simulink model "ADCSSimulator"  (R2024a)
settings: Solver=ode4  StartTime=0.0  StopTime=600  FixedStep=0.01  MaxStep=0.1  RelTol=1e-3  AbsTol=1e-3
values from neighbouring files (symbols this model uses):
  ActuatorAllocationMatrix = ActuatorPhysicalMatrix' * inv(ActuatorPhysicalMatrix * ActuatorPhysicalMatrix')    [set_Init.m]
  ActuatorPhysicalMatrix = [1, 0, 0, 0 ... (first row only)    [set_Init.m]
  albedo_irradiance = 300    [set_Init.m]
  b = 0    [set_Init.m]
  Cd = 2.2    [set_Init.m]
  h_bias = [0; 0; 0]    [set_Init.m]
  J = 4.0e-3 / 628    (= 6.36942675159e-06)    [set_Init.m]
  k_Bdot = ((4 * pi * 0.5236 * 0.0055) / (5677.2 * (4.5e-5)^2))    (= 3147.8423197)    [set_Init.m]
  K_E = K_T    (= 0.0022)    [set_Init.m]
  K_T = 0.0022    [set_Init.m]
  P0 = blkdiag(P0_att, P0_bias)    [set_Init.m]
  P0_att = eye(3) * initial_variance_rad2    [set_Init.m]
  PowerVoltageBus_01 = 3.3    [set_Init.m]
  PowerVoltageBus_02 = 3.3    [set_Init.m]
  PowerVoltageBus_03 = 3.3    [set_Init.m]
  PowerVoltageBus_04 = 3.3    [set_Init.m]
  PowerVoltageBus_05 = 3.3    [set_Init.m]
  PowerVoltageBus_06 = 3.3    [set_Init.m]
  PowerVoltageBus_07 = 3.3    [set_Init.m]
  PowerVoltageBus_08 = 3.3    [set_Init.m]
  PowerVoltageBus_09 = 3.3    [set_Init.m]
  PowerVoltageBus_10 = 3.3    [set_Init.m]
  PowerVoltageBus_11 = 3.3    [set_Init.m]
  PowerVoltageBus_12 = 0.0    (= 0)    [set_Init.m]
  PowerVoltageBus_13 = 0.0    (= 0)    [set_Init.m]
  PowerVoltageBus_14 = 0.0    (= 0)    [set_Init.m]
  PowerVoltageBus_15 = 0.0    (= 0)    [set_Init.m]
  R = 2.0    (= 2)    [set_Init.m]
  ressidual_m = [3e-4; -2e-4; 1e-4]    [set_Init.m]
  solar_irradiance = 1361    [set_Init.m]
  surface_areas = [A_xy, A_yz, A_xz, A_xy, A_yz, A_xz]    [set_Init.m]
  surface_normals_body = [eye(3) -eye(3)]    [set_Init.m]
  surface_positions_body = [       hx,   0,   0 ... (first row only)    [set_Init.m]
  surface_reflectivities = [0.9 0.8 0.9 0.9 0.9 0.9]    [set_Init.m]
  Switch_01 = 1    [set_Init.m]
  Switch_02 = 1    [set_Init.m]
  Switch_03 = 1    [set_Init.m]
  Switch_04 = 1    [set_Init.m]
  Switch_05 = 1    [set_Init.m]
  Switch_06 = 1    [set_Init.m]
  Switch_07 = 1    [set_Init.m]
  Switch_08 = 1    [set_Init.m]
  Switch_09 = 1    [set_Init.m]
  Switch_10 = 1    [set_Init.m]
  Switch_11 = 1    [set_Init.m]
  Switch_12 = 0    [set_Init.m]
  Switch_13 = 0    [set_Init.m]
  Switch_14 = 0    [set_Init.m]
  Switch_15 = 0    [set_Init.m]
  visSampleTime = 0.1    [set_Init.m]
undefined symbols (not defined in the file or in its folder): attitude, Controller, epoch, IAU, juliandate, Kd, km, Kp, m, rad, s, satellite, SGP4_parameters, simulator, UKF_parameters, WMM2020
libraries: sharedtransform x27, aerolibutil x22, aerolibconvert2 x18, simulink_extras x16, matrix_library x6, aerolibtransform2 x4, vrlib x2, aerolibgravity2 x2, aerolibobsolete x1, aerolibattitudesys x1, simulink x1
(part 8 of 8)

== matlab function ADCSSimulator/ADCS/ADCS Software/Orbit Detemination/UKF Orbit  ==
  data: is_reset_triggered input; initial_state input; initial_covariance input; gps_pos_ICRF input; r_est_ICRF output; dt input; Q input; R input; v_est_ICRF output; Bc_est output; satellite_mass_kg input; P_out output; is_healthy output
function [r_est_ICRF, v_est_ICRF, Bc_est, P_out, is_healthy] = ukf_orbit_estimator(is_reset_triggered, initial_state, initial_covariance, gps_pos_ICRF, dt, Q, R, satellite_mass_kg)
% ukf_orbit_estimator Estimates satellite orbit state using a 7-state UKF.
%
% Function Objective:
% This function is the primary, high-fidelity orbit estimator. It fuses a
% physics-based dynamics model with GPS measurements to produce an accurate
% and continuously updated state estimate. It includes a health flag to
% enable system-level fault detection.
%
% Key Features:
%   - 7-State Vector: [r, v, Bc] for adaptive drag estimation.
%   - Reset Mechanism: Allows re-initialization from a TLE.
%   - Health Monitoring: Outputs a flag indicating filter health.
%   - Advanced Dynamics: Includes J2 and atmospheric drag.
%
% Inputs:
%   is_reset_triggered: (boolean)  If true, reset filter to initial values.
%   initial_state:      (7x1 double) State for initialization [r, v, Bc].
%   initial_covariance: (7x7 double) Covariance for initialization.
%   gps_pos_ICRF:       (3x1 double) GPS position in ICRF [km]. Use NaN if invalid.
%   dt:                 (double)   Time step [s].
%   Q:                  (7x7 double) Process noise covariance.
%   R:                  (3x3 double) Measurement noise covariance.
%   satellite_mass_kg:  (double)   Satellite mass [kg].
%
% Outputs:
%   r_est_ICRF: (3x1 double) Estimated position [km].
%   v_est_ICRF: (3x1 double) Estimated velocity [km/s].
%   Bc_est:     (double)   Estimated ballistic coefficient [m^2/kg].
%   P_out:      (7x7 double) Final estimated covariance.
%   is_healthy: (boolean)  True if the filter is operating correctly.
%===============================================================================

    persistent x_est P;

    % --- Initialization and Reset Logic ---
    if isempty(x_est) || is_reset_triggered
        x_est = initial_state;
        P = initial_covariance;
    end

    % --- UKF Tuning Parameters ---
    n = 7; alpha = 1e-3; kappa = 0; beta = 2;
    lambda = alpha^2 * (n + kappa) - n;

    %===========================================================================
    % --- 1. PREDICTION STEP ---
    %===========================================================================
    sigma_points = zeros(n, 2*n + 1);
    sigma_points(:, 1) = x_est;
    
    % --- Cholesky Decomposition for Sigma Points ---
    % This is a critical health check. If P is not positive definite, the
    % filter has mathematically diverged.
    [P_sqrt, p] = chol((n + lambda) * P, 'lower');
    if p > 0
        % CRITICAL FAILURE: Report unhealthy and exit immediately.
        r_est_ICRF = x_est(1:3); v_est_ICRF = x_est(4:6);
        Bc_est = x_est(7); P_out = P;
        is_healthy = false; % This flag triggers the switch to SAFE mode.
        return;
    end
    
    for i = 1:n
        sigma_points(:, i+1)   = x_est + P_sqrt(:, i);
        sigma_points(:, i+n+1) = x_est - P_sqrt(:, i);
    end

    % --- Propagate Sigma Points through Non-Linear Dynamics ---
    propagated_sigma_points = zeros(n, 2*n + 1);
    for i = 1:(2*n + 1)
        propagated_sigma_points(:, i) = state_transition_function(sigma_points(:, i), dt, satellite_mass_kg);
    end

    % --- Calculate Predicted State and Covariance ---
    weights_m = [lambda/(n+lambda), 0.5/(n+lambda) * ones(1, 2*n)];
    weights_c = weights_m;
    weights_c(1) = weights_c(1) + (1 - alpha^2 + beta);
    
    x_priori = propagated_sigma_points * weights_m';
    
    P_priori = zeros(n, n);
    for i = 1:(2*n + 1)
        diff = propagated_sigma_points(:, i) - x_priori;
        P_priori = P_priori + weights_c(i) * (diff * diff');
    end
    P_priori = P_priori + Q;

    %===========================================================================
    % --- 2. UPDATE STEP ---
    %===========================================================================
    if ~any(isnan(gps_pos_ICRF))
        % Transform sigma points into measurement space (position only)
        z_sigma_points = propagated_sigma_points(1:3, :);
        z_pred = z_sigma_points * weights_m';

        % Calculate Innovation Covariance (S) and Cross-Covariance (T)
        S = zeros(3, 3); T = zeros(n, 3);
        for i = 1:(2*n + 1)
            z_diff = z_sigma_points(:, i) - z_pred;
            x_diff = propagated_sigma_points(:, i) - x_priori;
            S = S + weights_c(i) * (z_diff * z_diff');
            T = T + weights_c(i) * (x_diff * z_diff');
        end
        S = S + R;
        
        % Calculate Kalman Gain and update state/covariance
        K = T / S;
        innovation = gps_pos_ICRF - z_pred;
        x_est = x_priori + K * innovation;
        P = P_priori - K * S * K';
    else
        % No GPS data, so the prediction becomes the best estimate
        x_est = x_priori;
        P = P_priori;
    end
    
    % Enforce physical constraint on the ballistic coefficient
    if x_est(7) < 0, x_est(7) = 0; end

    % --- Final Output ---
    r_est_ICRF = x_est(1:3);
    v_est_ICRF = x_est(4:6);
    Bc_est     = x_est(7);
    P_out      = P;
    is_healthy = true; % If we reached this point, the filter is healthy.
end

% --- Sub-function: State Transition (Dynamics Integration) ---
function x_next = state_transition_function(x, dt, m)
    k1 = dynamics(x, m);
    k2 = dynamics(x + 0.5*dt*k1, m);
    k3 = dynamics(x + 0.5*dt*k2, m);
    k4 = dynamics(x + dt*k3, m);
    x_next = x + (dt/6)*(k1 + 2*k2 + 2*k3 + k4);
end

% --- Sub-function: Equations of Motion ---
function dxdt = dynamics(x, m)
    r_vec = x(1:3); v_vec = x(4:6); Bc = x(7);
    r_norm = norm(r_vec);
    
    % --- Physical Constants ---
    mu = 398600.4418; J2 = 0.00108263; R_earth = 6378.137;
    
    % --- Gravitational Model ---
    a_2body = -mu * r_vec / r_norm^3;
    pre = -1.5 * mu * J2 * R_earth^2 / r_norm^5;
    z_factor = 5 * (r_vec(3)/r_norm)^2;
    a_j2 = [pre * r_vec(1) * (1 - z_factor);
            pre * r_vec(2) * (1 - z_factor);
            pre * r_vec(3) * (3 - z_factor)];
            
    % --- Atmospheric Drag Model ---
    alt_km = r_norm - R_earth;
    rho = atmospheric_density_model(alt_km); % kg/m^3
    
    we = 7.292115e-5; % Earth rotation rate [rad/s]
    v_rel_m_s = (v_vec - cross([0; 0; we], r_vec)) * 1000; % to m/s
    v_rel_norm = norm(v_rel_m_s);
    
    a_drag_m_s2 = -0.5 * Bc * rho * v_rel_norm * v_rel_m_s;
    a_drag_km_s2 = a_drag_m_s2 / 1000; % to km/s^2
    
    a_total = a_2body + a_j2 + a_drag_km_s2;
    
    % The derivative of Bc is modeled as zero (a random walk)
    dxdt = [v_vec; a_total; 0];
end

% --- Sub-function: Atmospheric Density Model ---
function rho = atmospheric_density_model(alt_km)
    % Simple exponential atmospheric density model.
    % NOTE: For a high-fidelity thesis, replacing this with a standard model
    % (e.g., NRLMSISE-00) would be a major enhancement.
    h0 = 400; rho0 = 2.4e-12; H = 55;
    rho = rho0 * exp(-(alt_km - h0) / H);
end

== matlab function ADCSSimulator/ADCS/ADCS Software/Attitude Determination/Attitude Estimation Algorithm (MEKF)/MATLAB Function9 ==
  data: q_est output; P_est output; q_feedback input; P_feedback input; q_quest input; P_quest_attitude input; lambda_max_quest input; gyro_meas input; b_sun input; b_mag input; r_sun input; r_mag input; dt input; Q_noise input; R_sun input; R_mag input; reset_threshold input
function [q_est, P_est] = attitude_mekf_simplified( ...
    q_feedback, P_feedback, ...
    q_quest, P_quest_attitude, lambda_max_quest, ...
    gyro_meas, b_sun, b_mag, r_sun, r_mag, ...
    dt, Q_noise, R_sun, R_mag, reset_threshold)
% ATTITUDE_EKF_SIMPLIFIED (Quaternion Estimation Only)
%
% This is a simplified, robust MEKF that only estimates the attitude.
% It uses a safe initialization and robustly hybridizes with QUEST
% solutions when they are available and of high quality.
%
% UNIT CONVENTION
% Attitude Error State & Covariance: milli-radians (mrad)
% Gyro Measurement:                milli-radians/second (mrad/s)
% Magnetic Field Measurement:      micro-Tesla (uT)
%
% Sun Sensor Noise R_sun:          radians^2 (rad^2)
% Mag Sensor Noise R_mag:          micro-Tesla^2 (uT^2)
% Process Noise Q_noise (3x3):     (mrad/s)^2
% =========================================================================
% 0) INITIALIZATION & HYBRIDIZATION
% =========================================================================
LAMBDA_THRESHOLD = 0.999;
is_sun_available = ~any(isnan(b_sun));
is_quest_valid = is_sun_available && ~any(isnan(q_quest)) && (lambda_max_quest > LAMBDA_THRESHOLD);

% Check if this is the first run of the simulation
is_first_run = (norm(q_feedback) < 1e-6);

if is_first_run
    % On the first run, ALWAYS initialize with a default attitude and
    % a very large uncertainty to ensure a safe start.
    q_prev = [1; 0; 0; 0];
    P_prev = eye(3) * 1e9; % Huge uncertainty: (1e6 mrad)^2
else
    % Standard Operation: Check for Reset
    perform_reset = false;
    if is_quest_valid
        % Only reset if the MEKF is more uncertain than a fresh QUEST solution
        if trace(P_feedback) > trace(P_quest_attitude) && trace(P_feedback) > reset_threshold
            perform_reset = true;
        end
    end

    if perform_reset
        % Reset the state using the high-quality QUEST solution
        q_prev = q_quest;
        P_prev = P_quest_attitude;
    else
        % No reset, continue propagating the filter's own estimate
        q_prev = q_feedback;
        P_prev = P_feedback;
    end
end

% =========================================================================
% 1) PREDICTION
% =========================================================================
omega = gyro_meas; % No bias estimation
q_pred = propagate_with_gyro_expmap(q_prev, omega, dt);

% State is 3x1 (d_theta), so Fx is 3x3
Fx = -skew_symmetric(omega / 1000); % Convert mrad/s to rad/s for kinematics
F = expm(Fx * dt);

P_pred = F * P_prev * F' + Q_noise;
P_pred = 0.5 * (P_pred + P_pred'); % Enforce symmetry

% =========================================================================
% 2) BATCH UPDATE
% =========================================================================
q_est = q_pred;
P_est = P_pred;

H_stack = zeros(6,3);
y_stack = zeros(6,1);
R_stack = zeros(6,6);
num_valid = 0;
C_pred = quat2rotm(q_pred');

% Sun Sensor Measurement
if is_sun_available
    num_valid = num_valid + 1;
    idx = 1:3;
    b_pred_sun = C_pred * r_sun;
    y_sun      = b_sun - b_pred_sun;
    H_sun      = skew_symmetric(b_pred_sun) / 1000; % Maps d(theta)_mrad to d(y)_rad

    H_stack(idx,:) = H_sun;
    y_stack(idx)   = y_sun;
    R_stack(idx,idx) = R_sun;
end

% Magnetometer Measurement
if ~any(isnan(b_mag))
    num_valid = num_valid + 1;
    idx = (num_valid-1)*3 + (1:3);
    b_pred_mag = C_pred * r_mag;
    y_mag      = b_mag - b_pred_mag;
    H_mag      = skew_symmetric(b_pred_mag) / 1000; % Maps d(theta)_mrad to d(y)_uT

    H_stack(idx,:)   = H_mag;
    y_stack(idx)     = y_mag;
    R_stack(idx,idx) = R_mag;
end

% Perform Update
if num_valid > 0
    m = num_valid*3;
    H = H_stack(1:m,:);
    y = y_stack(1:m,:);
    R = R_stack(1:m,1:m);

    S = H*P_pred*H' + R;
    S = 0.5*(S + S');

    K = (P_pred*H') / S;

    dtheta_mrad = K * y;
    dtheta_rad = dtheta_mrad / 1000;

    dq = [1; 0.5*dtheta_rad];
    dq = dq / norm(dq);

    q_est = quat_multiply(q_pred, dq);

    I_KH = eye(3) - K*H;
    P_est = I_KH*P_pred*I_KH' + K*R*K';
    P_est = 0.5*(P_est + P_est');
end

q_est = q_est / norm(q_est);

end

% =========================================================================
% Helper Functions
% =========================================================================
function q_out = propagate_with_gyro_expmap(q_prev, omega_mrad_s, dt)
    omega_rad_s = omega_mrad_s / 1000;
    theta = norm(omega_rad_s) * dt;
    if theta > 1e-9
        axis = omega_rad_s / (theta/dt);
        half = 0.5*theta;
        dq = [cos(half); axis * sin(half)];
        q_out = quat_multiply(q_prev, dq);
    else
        q_out = q_prev;
    end
    q_out = q_out / norm(q_out);
end

function C = skew_symmetric(v)
    C = [   0   -v(3)  v(2);
          v(3)    0   -v(1);
         -v(2)  v(1)    0  ];
end

function q_out = quat_multiply(q1, q2)
    w1 = q1(1); v1 = q1(2:4);
    w2 = q2(1); v2 = q2(2:4);
    w  = w1*w2 - dot(v1,v2);
    v  = w1*v2 + w2*v1 + cross(v1,v2);
    q_out = [w; v];
end

== matlab function ADCSSimulator/ADCS/ADCS Software/MATLAB Function2 ==
  data: p input; trace_p output
function trace_p = Trace(p)

trace_p = trace(p);

== matlab function ADCSSimulator/ADCS/ADCS Software/Orbit Detemination/UKF Orbit Estimator ==
  settings: updateMethod=DISCRETE
  data: r_meas input; r_est output; dt input; v_est output; Q input; R input; P_out output
function [r_est, v_est, P_out] = ukf_orbit_simple(r_meas, dt, Q, R)
% UKF orbit estimator (position only as measurement)
% 6-state UKF: [r; v]

persistent x_est P

n = 6; alpha = 1e-3; kappa = 0; beta = 2;
lambda = alpha^2*(n+kappa)-n;

% Initialize persistent state
if isempty(x_est)
    x_est = [r_meas; zeros(3,1)];
    P = eye(6)*1e4;
end

% Sigma points
sigma_pts = zeros(n,2*n+1);
sigma_pts(:,1) = x_est;
[P_sqrt, p] = chol((n+lambda)*P,'lower');
if p>0
    P_sqrt = sqrt(n+lambda)*eye(n);
end
for i=1:n
    sigma_pts(:,i+1)   = x_est + P_sqrt(:,i);
    sigma_pts(:,i+n+1) = x_est - P_sqrt(:,i);
end

% Propagate sigma points
prop_sigma = zeros(n,2*n+1);
for i=1:2*n+1
    prop_sigma(:,i) = rk4_orbit(sigma_pts(:,i), dt);
end

% Predicted state and covariance
wm = [lambda/(n+lambda) repmat(0.5/(n+lambda),1,2*n)];
wc = wm; wc(1) = wc(1)+(1-alpha^2+beta);

x_priori = prop_sigma*wm';
P_priori = zeros(n);
for i=1:2*n+1
    diff = prop_sigma(:,i)-x_priori;
    P_priori = P_priori + wc(i)*(diff*diff');
end
P_priori = P_priori + Q;

% Measurement update
if ~any(isnan(r_meas))
    Z = prop_sigma(1:3,:);
    z_pred = Z*wm';
    
    S = zeros(3); T = zeros(n,3);
    for i=1:2*n+1
        dz = Z(:,i)-z_pred;
        dx = prop_sigma(:,i)-x_priori;
        S = S + wc(i)*(dz*dz');
        T = T + wc(i)*(dx*dz');
    end
    S = S + R;
    K = T/S;
    x_est = x_priori + K*(r_meas - z_pred);
    P = P_priori - K*S*K';
else
    x_est = x_priori;
    P = P_priori;
end

r_est = x_est(1:3);
v_est = x_est(4:6);
P_out = P;

end

%% RK4 integrator
function x_next = rk4_orbit(x, dt)
r = x(1:3); v = x(4:6);

k1 = orbit_dynamics(r,v);
k2 = orbit_dynamics(r + 0.5*dt*k1(1:3), v + 0.5*dt*k1(4:6));
k3 = orbit_dynamics(r + 0.5*dt*k2(1:3), v + 0.5*dt*k2(4:6));
k4 = orbit_dynamics(r + dt*k3(1:3), v + dt*k3(4:6));

r_next = r + dt/6*(k1(1:3)+2*k2(1:3)+2*k3(1:3)+k4(1:3));
v_next = v + dt/6*(k1(4:6)+2*k2(4:6)+2*k3(4:6)+k4(4:6));

x_next = [r_next; v_next];
end

%% Orbital dynamics (gravity + J2)
function dx = orbit_dynamics(r,v)
mu = 3.986004418e14; Re = 6378137; J2 = 1.08263e-3;
r_norm = norm(r);
a_grav = -mu*r/r_norm^3;

% J2 perturbation
rx=r(1); ry=r(2); rz=r(3); z2=rz^2;
fac = 1.5*J2*mu*Re^2/r_norm^5;
a_j2 = fac * [rx*(5*z2/r_norm^2 - 1); ry*(5*z2/r_norm^2 - 1); rz*(5*z2/r_norm^2 -3)];

dx = [v; a_grav + a_j2];
end

== matlab function ADCSSimulator/ADCS/ADCS Software/Attitude Control/Chart/Nadir_Pointing/َAttitude Controller (LQR Controller)/PD Quaternion Feedback Controller/Dipole Smoother00 ==
  data: B input; m output; T_c input; k input
function m = computeMagneticDipole(B, T_c, k)
    % Computes the magnetic dipole moment (m) given:
    % B: Geomagnetic field vector in body frame [3x1] (T)
    % Tc: Commanded control torque in body frame [3x1] (N·m)
    % k: Regularization constant (scalar)
    %
    % Output:
    % m: Magnetic dipole moment in body frame [3x1] (A·m^2)

    % Validate inputs
    if length(B) ~= 3 || length(T_c) ~= 3
        error('B and Tc must be 3x1 vectors.');
    end

    % Create the skew-symmetric matrix of B
    B_mat = [
        0,       B(3),  -B(2);
       -B(3),   0,       B(1);
        B(2),  -B(1),    0
    ];

    % Compute the SR-Inverse
    I = eye(3); % 3x3 identity matrix
    regularized_inverse = inv((B_mat.' * B_mat + k * I)) / B_mat.';

    % Compute the magnetic dipole moment
    m = regularized_inverse * T_c;
end

== matlab function ADCSSimulator/ADCS/ADCS Software/Orbit Detemination/Mode Manager2 ==
  data: r_true input; error_vec output; r_est input; RMS_error output; mean_error output
function [error_vec, RMS_error, mean_error] = evaluate_position_error(r_true, r_est)
% evaluate_position_error Computes the estimation error of satellite position
%
% Inputs:
%   r_true - Nx3 matrix of true satellite positions [m]
%   r_est  - Nx3 matrix of estimated satellite positions [m]
%
% Outputs:
%   error_vec  - Nx1 vector of position errors (Euclidean distance) [m]
%   RMS_error  - Root-mean-square error over all samples [m]
%   mean_error - Mean absolute error over all samples [m]

    % Ensure same size
    if size(r_true,1) ~= size(r_est,1)
        error('r_true and r_est must have the same number of samples.');
    end

    % Vector of Euclidean errors
    error_vec = sqrt(sum((r_true - r_est).^2, 2));

    % RMS error
    RMS_error = sqrt(mean(error_vec.^2));

    % Mean absolute error
    mean_error = mean(error_vec);
end

== matlab function ADCSSimulator/ADCS/ADCS Software/Orbit Detemination/UKF Orbit Estimator1 ==
  data: gps_pos_ICRF input; r_est output; dt input; v_est output; Q_in input; R_in input; init_flag input; x0 input; P0 input; P_out output; is_healthy output
function [r_est, v_est, P_out, is_healthy] = ukf_orbit_block(gps_pos_ICRF, dt, Q_in, R_in, init_flag, x0, P0)
% UKF_ORBIT_BLOCK - 6-state UKF for ICRF orbit (2-body + J2 + drag + SRP)
% Inputs:
%  gps_pos_ICRF : 3x1 measured position [m] (use NaN to skip update)
%  dt            : timestep [s]
%  Q_in          : 6x6 process noise covariance (optional; pass [] to use default)
%  R_in          : 3x3 measurement noise covariance (optional; pass [] to use default)
%  init_flag     : boolean, true => initialize with x0 and P0
%  x0            : 6x1 initial state [r0; v0] (required if init_flag true)
%  P0            : 6x6 initial covariance (optional)
% Outputs:
%  r_est, v_est, P_out, is_healthy

    persistent x_est P params ukf_initialized

    % -------------------- default physical params (SI) --------------------
    if isempty(params)
        params.mu     = 3.986004418e14;   % m^3/s^2
        params.Re     = 6378137.0;        % m
        params.J2     = 1.08263e-3;
        params.omegaE = 7.2921150e-5;     % rad/s

        % CubeSat example
        params.m  = 4.0;   % kg
        params.A  = 0.03;  % m^2
        params.Cd = 2.2;
        params.Cr = 1.3;

        % SRP
        params.Psrp  = 4.56e-6;           % N/m^2
        params.r_sun = [1.496e11; 0; 0];  % approx 1 AU along +x

        % atmosphere exponential baseline (around 400 km)
        params.rho0 = 2.4e-12;  % kg/m^3 at h0
        params.h0   = 400e3;    % m
        params.H    = 55e3;     % m
    end

    % -------------------- defaults for Q, R, P0 --------------------
    default_P0 = diag([100^2,100^2,100^2, 0.1^2,0.1^2,0.1^2]);
    default_Q  = diag([1e-4,1e-4,1e-4, 1e-8,1e-8,1e-8]);
    default_R  = diag([15^2,15^2,15^2]);

    if isempty(Q_in)
        Q = default_Q;
    else
        Q = Q_in;
    end
    if isempty(R_in)
        R = default_R;
    else
        R = R_in;
    end

    % -------------------- UKF tuning --------------------
    n = 6;
    alpha = 1e-2; beta = 2; kappa = 0;
    lambda = alpha^2*(n + kappa) - n;
    c = n + lambda;
    Wm = zeros(2*n+1,1); Wc = zeros(2*n+1,1);
    Wm(1) = lambda / c; Wc(1) = Wm(1) + (1 - alpha^2 + beta);
    Wm(2:end) = 1/(2*c); Wc(2:end) = 1/(2*c);

    % -------------------- initialization --------------------
    if isempty(ukf_initialized) || init_flag
        if init_flag
            if nargin < 6 || isempty(x0) || numel(x0)~=6
                error('init_flag true requires x0 (6x1).');
            end
            x_est = x0(:);
        else
            % first call without explicit init -> try init from gps_pos_ICRF
            if any(isnan(gps_pos_ICRF))
                error('First call requires valid gps_pos_ICRF or init_flag=true with x0.');
            end
            r0 = gps_pos_ICRF(:);
            rnorm = norm(r0) + 1e-12;
            % approximate circular speed and direction (tangent)
            vmag = sqrt(params.mu / rnorm);
            % choose a stable perpendicular vector
            k = [0;0;1];
            t = cross(k, r0);
            if norm(t) < 1e-6
                t = cross([1;0;0], r0);
            end
            t = t / norm(t);
            v0 = vmag * t;
            x_est = [r0; v0];
        end
        if nargin>=7 && ~isempty(P0)
            P = P0;
        else
            P = default_P0;
        end
        ukf_initialized = true;
    end

    is_healthy = true;

    % -------------------- ensure shapes --------------------
    gps_pos_ICRF = gps_pos_ICRF(:);
    if numel(gps_pos_ICRF)~=3
        error('gps_pos_ICRF must be 3x1 (or NaN).');
    end

    % -------------------- 1) sigma points --------------------
    P = 0.5*(P + P.');  % symmetrize
    try
        A = chol(c * P, 'lower'); % A*A' = cP
    catch
        % regularize and retry
        epsfix = 1e-9 * eye(n);
        try
            A = chol(c * (P + epsfix), 'lower');
        catch
            % catastrophic -> soft reset if measurement available
            is_healthy = false;
            if ~any(isnan(gps_pos_ICRF))
                % reinit with measurement pos and approximate vel
                r0 = gps_pos_ICRF(:);
                rnorm = norm(r0) + 1e-12;
                vmag = sqrt(params.mu / rnorm);
                k = [0;0;1];
                t = cross(k, r0);
                if norm(t) < 1e-6, t = cross([1;0;0], r0); end
                t = t / norm(t);
                x_est = [r0; vmag*t];
                P = default_P0;
                r_est = x_est(1:3); v_est = x_est(4:6); P_out = P;
                return
            else
                r_est = x_est(1:3); v_est = x_est(4:6); P_out = P;
                return
            end
        end
    end

    X = zeros(n, 2*n+1);
    X(:,1) = x_est;
    for i=1:n
        X(:,i+1)   = x_est + A(:,i);
        X(:,i+1+n) = x_est - A(:,i);
    end

    % -------------------- 2) propagate sigma points (RK4) --------------------
    Xprop = zeros(size(X));
    for i=1:size(X,2)
        Xprop(:,i) = propagate_rk4(X(:,i), dt, params);
    end

    % -------------------- 3) predicted mean & covariance --------------------
    x_pred = Xprop * Wm;
    P_pred = zeros(n);
    for i=1:2*n+1
        dx = Xprop(:,i) - x_pred;
        P_pred = P_pred + Wc(i) * (dx * dx.');
    end
    P_pred = P_pred + Q;

    % -------------------- 4) measurement update (position only) --------------------
    if ~any(isnan(gps_pos_ICRF))
        z = gps_pos_ICRF(:);
        Zsig = Xprop(1:3, :);
        z_pred = Zsig * Wm;

        S = zeros(3);
        Pxz = zeros(n,3);
        for i=1:2*n+1
            dz = Zsig(:,i) - z_pred;
            dx = Xprop(:,i) - x_pred;
            S = S + Wc(i) * (dz * dz.');
            Pxz = Pxz + Wc(i) * (dx * dz.');
        end
        S = S + R;

        % Kalman gain
        K = Pxz / S;
        innov = z - z_pred;

        % gating (simple)
        nis = innov' * (S\innov);
        gating_thresh = 16; % ~ chi2inv(0.995,3) ~ 12.84 ; use small margin
        if nis > 1e6
            % catastrophic innovation: skip update, mark unhealthy
            x_est = x_pred;
            P = P_pred;
            is_healthy = false;
        elseif nis > gating_thresh
            % large innovation: reject update (keep prediction)
            x_est = x_pred;
            P = P_pred;
            is_healthy = false;
        else
            x_est = x_pred + K * innov;
            P = P_pred - K * S * K.';
        end
    else
        x_est = x_pred;
        P = P_pred;
    end

    % -------------------- postprocess P --------------------
    P = 0.5*(P + P.');
    % small eigen-clamp to remove numerical negative eigenvalues
    [V,D] = eig(P);
    d = diag(D);
    d(d < 0) = 0;
    P = V * diag(d) * V.';

    % basic health checks
    if any(isnan(x_est)) || any(isnan(P(:))) || ~isreal(P)
        is_healthy = false;
    end
    if trace(P) > 1e14
        is_healthy = false;
        if ~any(isnan(gps_pos_ICRF))
            % soft reset
            r0 = gps_pos_ICRF(:);
            rnorm = norm(r0) + 1e-12;
            vmag = sqrt(params.mu / rnorm);
            k = [0;0;1];
            t = cross(k, r0);
            if norm(t) < 1e-6, t = cross([1;0;0], r0); end
            t = t / norm(t);
            x_est = [r0; vmag*t];
            P = default_P0;
        end
    end

    % outputs
    r_est = x_est(1:3);
    v_est = x_est(4:6);
    P_out = P;
end

% -------------------- RK4 propagate --------------------
function xnext = propagate_rk4(x, dt, params)
    k1 = eom(x, params);
    k2 = eom(x + 0.5*dt*k1, params);
    k3 = eom(x + 0.5*dt*k2, params);
    k4 = eom(x + dt*k3, params);
    xnext = x + (dt/6)*(k1 + 2*k2 + 2*k3 + k4);
end

% -------------------- equations of motion --------------------
function dxdt = eom(x, params)
    r = x(1:3);
    v = x(4:6);
    rnorm = norm(r) + 1e-12;

    % 2-body
    a2b = -params.mu * r / (rnorm^3);

    % J2
    z = r(3);
    r2 = rnorm^2;
    r5 = rnorm^5;
    factor = -1.5 * params.J2 * params.mu * params.Re^2 / r5;
    aJ2 = factor * [ r(1) * (1 - 5*(z^2)/r2);
                     r(2) * (1 - 5*(z^2)/r2);
                     r(3) * (3 - 5*(z^2)/r2) ];

    % atmosphere (exponential)
    alt = rnorm - params.Re;
    rho = rho_exp(alt, params);

    % relative velocity (assume atmosphere rotates with Earth)
    omega = [0;0;params.omegaE];
    v_rel = v - cross(omega, r);
    vrel_norm = norm(v_rel) + 1e-12;

    % drag (m/s^2)
    a_drag = -0.5 * (params.Cd * params.A / params.m) * rho * vrel_norm * v_rel;

    % SRP (no eclipse model)
    d = params.r_sun - r;
    a_srp = (params.Psrp * params.Cr * params.A / params.m) * (d / (norm(d)+1e-12));

    a_total = a2b + aJ2 + a_drag + a_srp;

    dxdt = [v; a_total];
end

% -------------------- exponential atmosphere --------------------
function rho = rho_exp(alt, params)
    if alt < -1e4, alt = -1e4; end
    rho = params.rho0 * exp(-(alt - params.h0) / params.H);
    if rho < 1e-20, rho = 1e-20; end
end

== matlab function ADCSSimulator/ADCS/ADCS Software/Orbit Detemination/Mode Manager ==
  data: ukf_is_healthy input; is_nominal_mode output; ground_reset_cmd input; trigger_ukf_reset output
function [is_nominal_mode, trigger_ukf_reset] = mode_manager(ukf_is_healthy, ground_reset_cmd)
    persistent in_nominal_mode;
    if isempty(in_nominal_mode)
        in_nominal_mode = true; % Start in NOMINAL mode
    end

    % FDIR State Machine Logic
    if in_nominal_mode
        if ~ukf_is_healthy
            % FAULT DETECTED: UKF has failed. Transition to SAFE mode.
            in_nominal_mode = false;
        end
    else % We are in SAFE mode
        if ground_reset_cmd
            % RECOVERY: Ground commands a reset. Transition to NOMINAL.
            in_nominal_mode = true;
        end
    end

    % Determine if a reset should be triggered THIS time step
    trigger_ukf_reset = ground_reset_cmd;

    is_nominal_mode = in_nominal_mode;
end

== matlab function ADCSSimulator/EPS/EPS HouseKeeping/SOC Calculator/MATLAB Function ==
  data: E_used input; SOC output; E_capacity input
function SOC = SOC(E_used, E_capacity)
SOC = max(0, min(100, (1 - E_used / E_capacity) * 100));
end

== matlab function ADCSSimulator/ADCS/ADCS Software/Attitude Control/Chart/Nadir_Pointing/َAttitude Controller (LQR Controller)/PD Quaternion Feedback Controller/Torque to Dipole Converter ==
  data: B_body input; torque_cmd_body input; dipole_cmd_body output
function dipole_cmd_body = calculateMTQDipole(B_body, torque_cmd_body)
% calculateMTQDipole Converts a commanded torque to a commanded dipole moment.
%
% This function takes the desired torque from a controller and the local
% magnetic field vector to calculate the required magnetic dipole moment
% for the magnetorquers (MTQs).
%
% It inherently handles the physical limitation that torque cannot be
% generated parallel to the magnetic field.
%
% Inputs:
%   tau_cmd_body: 3x1 vector of the commanded torque in the body frame (N*m)
%   B_body:       3x1 vector of the magnetic field in the body frame (Tesla)
%
% Output:
%   m_cmd_body:   3x1 vector of the commanded magnetic dipole moment (A*m^2)

    % Calculate the squared magnitude of the magnetic field
    B_sq = dot(B_body, B_body);

    % Prevent division by zero if the magnetic field is negligible
    if B_sq < 1e-12 % (equivalent to a field of 1 nT)
        dipole_cmd_body = [0; 0; 0];
        return;
    end
    
    % Calculate the required dipole moment.
    % The formula m = cross(B, tau) / ||B||^2 finds the dipole that
    % generates the component of tau perpendicular to B. The component of
    % tau parallel to B is automatically ignored by the cross product.
    dipole_cmd_body = cross(B_body, torque_cmd_body) / B_sq;

end

== matlab function ADCSSimulator/ADCS/ADCS Software/Quaternion Error (deg)1 ==
  data: q_true input; error_angle_deg output; q_est input
function error_angle_deg = quaternion_angle_error(q_true, q_est)
% Calculates the angular error between two quaternions

% Inputs:
%   q_true: 4x1 true attitude quaternion [scalar; vector].
%   q_est:  4x1 estimated attitude quaternion [scalar; vector].
%
% Output:
%   error: 180-deg error.

    % Validate input dimensions.
    if ~isequal(size(q_true), [4,1]) || ~isequal(size(q_est), [4,1])
        error('Input quaternions must be 4x1 column vectors.');
    end

    % Step 1: Calculate the Error Quaternion
    % The error quaternion (delta_q) represents the rotation needed to get
    % from the estimated attitude to the true attitude.
    delta_q = quat_multiply(q_true, quat_inverse(q_est));

    % Step 2: Extract the Angular Error
    % The angle of rotation is calculated from the scalar part of the error
    % quaternion. The absolute value ensures we get the shortest path (<= 180 deg).
    scalar_part = abs(delta_q(1));
    
    % Clamp the value to 1.0 to prevent numerical errors from acos().
    scalar_part = min(1.0, scalar_part);
    
    error_angle_rad = 2 * acos(scalar_part);
    
    % Step 3: Convert to deg
    % Convert the angular error in degrees
    error_angle_deg = error_angle_rad * (180 / pi);
end

% Helper Functions for Quaternion Math
function q_out = quat_multiply(q1, q2)
    % Multiplies two quaternions, q1 * q2.
    s1 = q1(1); v1 = q1(2:4);
    s2 = q2(1); v2 = q2(2:4);
    
    s_out = s1*s2 - dot(v1, v2);
    v_out = s1*v2 + s2*v1 + cross(v1, v2);
    
    q_out = [s_out; v_out];
    % Re-normalize to prevent accumulation of floating-point errors.
    if norm(q_out) > 1e-9
        q_out = q_out / norm(q_out);
    else
        q_out = [1; 0; 0; 0]; % Return identity if result is zero
    end
end

function q_inv = quat_inverse(q)
    % The inverse of a unit quaternion is its conjugate.
    q_inv = [q(1); -q(2:4)];
end

== matlab function ADCSSimulator/ADCS/Environment Model/Orbit Eclipse Calculator/MATLAB Function1 ==
  data: r_sat input; isInEclipse output; r_sun input
function isInEclipse = checkEclipse(r_sat, r_sun)
    % Constants
    R_E = 6378137; % Earth's radius in m
    
    % Vector from satellite to Sun
    d = r_sat - r_sun;
    
    % Condition 1: Satellite behind Earth (relative to the Sun)
    condition1 = dot(r_sun, r_sat) < 0;
    
    % Perpendicular distance to Earth's shadow axis
    d_perp = norm(cross(r_sat, r_sun)) / norm(r_sun);
    
    % Earth's shadow radius at satellite's distance
    Rs = R_E * norm(r_sun) / (norm(r_sun) - R_E);
    
    % Condition 2: Satellite within Earth's shadow cone
    condition2 = d_perp < Rs;
    
    % Output: In eclipse or not
    InEclipse = condition1 && condition2;
    if InEclipse == 1
        isInEclipse = 1;
    else
        isInEclipse = 0;

end

== matlab function ADCSSimulator/ADCS/Environment Model/Disturbance Calculator/Aerodynamic Torque/MATLAB Function1 ==
  data: R_body input; aerodynamic_drag_torque output; V_body input; surface_normals input; surface_areas input; surface_positions input; Cd input
function aerodynamic_drag_torque = AerodynamicsDragTorque(R_body, V_body, ...
    surface_normals, surface_areas, surface_positions, Cd)
%AERODYNAMICSDRAGTORQUE Computes aerodynamic drag torque in body frame

% Inputs:
%   R_body            : [3x1] Satellite position vector in body frame [m]
%   V_body            : [3x1] Satellite velocity vector in body frame [m/s]
%   surface_normals   : [3x6] Unit normal vectors of each face in body frame
%   surface_areas     : [1x6] Area of each surface [m^2]
%   surface_positions : [3x6] Position vectors from CoM to surface center [m]
%   Cd                : [scalar] Drag coefficient

% Output:
%   aerodynamic_drag_torque : [3x1] Aerodynamic drag torque in body frame [Nm]

% Atmospheric model parameters
rho0 = 3.614e-14;  % [kg/m³]
h0 = 700;          % [km]
H = 88.667;        % [km]
Re_km = 6371;      % [km]

% Altitude from Earth's center
altitude_km = norm(R_body) * 1e-3 - Re_km;
rho = rho0 * exp(-(altitude_km - h0) / H);  % [kg/m^3]

% Relative velocity
V_rel = V_body;
V_rel_mag = norm(V_rel);

% Return zero torque if velocity is zero
if V_rel_mag == 0
    aerodynamic_drag_torque = zeros(3, 1);
    return;
end

% Normalize direction of velocity
V_rel_dir = V_rel / V_rel_mag;

% Initialize drag force matrix
F_drag = zeros(3, 6);

for i = 1:6
    n_i = surface_normals(:, i);
    dot_proj = dot(n_i, V_rel_dir);
    
    if dot_proj > 0
        A_proj = surface_areas(i) * dot_proj;
        F_i = -0.5 * rho * Cd * V_rel_mag^2 * A_proj * V_rel_dir;
        F_drag(:, i) = F_i;
    end
end

% Compute torques and total
torques = cross(surface_positions, F_drag);
aerodynamic_drag_torque = sum(torques, 2);

end
